simulink library "quatAttitudeController_lib"  (R2018b)
settings: Solver=VariableStepAuto  StartTime=0.0  StopTime=10.0  RelTol=1e-3
undefined symbols (not defined in the file or in its folder): quad
settings Model: Creator=fabian  LastModifiedBy=yannic

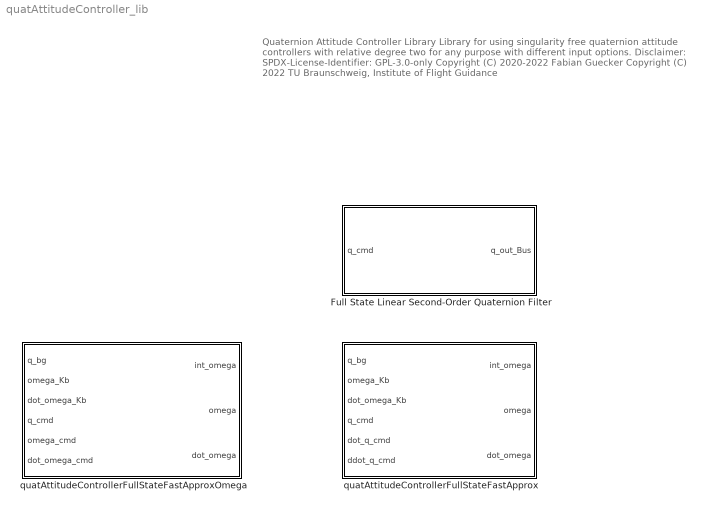
== system quatAttitudeController_lib ==
  note: Quaternion Attitude Controller Library
      |
      | Library for using singularity free quaternion attitude controllers with relative degree two
      | for any purpose with different input options.
      |
      | Disclaimer:
      | SPDX-License-Identifier: GPL-3.0-only
      |
      | Copyright (C) 2020-2022 Fabian Guecker
      | Copyright (C) 2022 TU Braunschweig, Institute of Flight Guidance
  Full State Linear Second-Order Quaternion Filter : Subsystem  mask{omega_0=200, D=1, q_0=[1; 0; 0; 0], omega_Kb_0=[0; 0; 0]}
      mask prompts: omega_0 "Natural frequency"; D "Damping factor"; q_0 "Inital quaternion"; omega_Kb_0 "Inital angular velocity"
  quatAttitudeControllerFullStateFastApprox : MATLAB Function  TreatAsAtomicUnit=on
  quatAttitudeControllerFullStateFastApproxOmega : MATLAB Function  TreatAsAtomicUnit=on

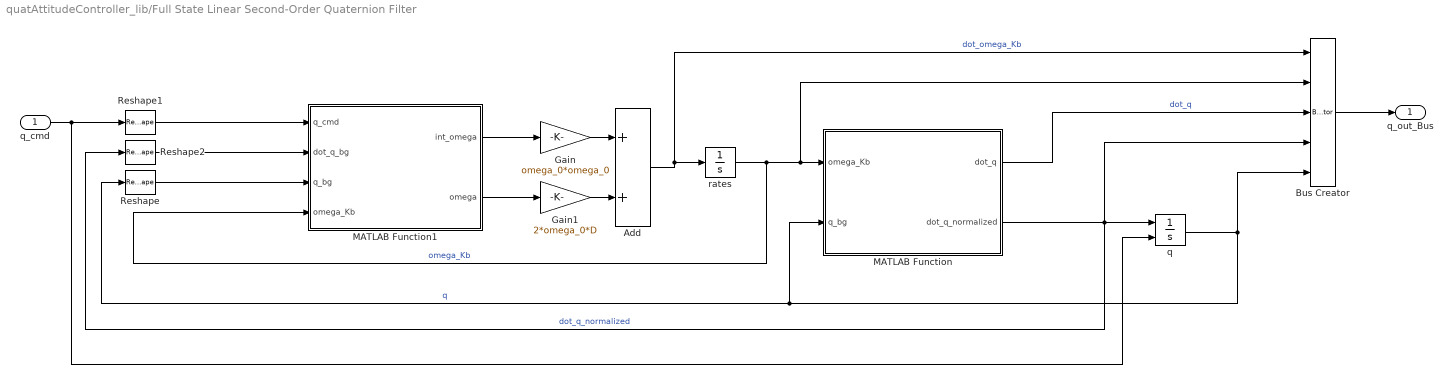
== system quatAttitudeController_lib/Full State Linear Second-Order Quaternion Filter ==
  q_cmd : Inport
  Add : Sum
  Bus Creator : BusCreator  Inputs=5
  Gain : Gain  Gain=omega_0*omega_0
  Gain1 : Gain  Gain=2*omega_0*D
  MATLAB Function : MATLAB Function  TreatAsAtomicUnit=on
  MATLAB Function1 : MATLAB Function  TreatAsAtomicUnit=on
  Reshape : Reshape  OutputDimensionality=Column vector (2-D)
  Reshape1 : Reshape  OutputDimensionality=Column vector (2-D)
  Reshape2 : Reshape  OutputDimensionality=Column vector (2-D)
  q : Integrator  InitialConditionSource=external  InitialCondition=q_0  UpperSaturationLimit=[inf;inf;-quad.z_s]  LowerSaturationLimit=[-inf;-inf;-inf]  ContinuousStateAttributes='quaternion'
  rates : Integrator  InitialCondition=omega_Kb_0  ContinuousStateAttributes='rates'
  q_out_Bus : Outport
  wires:
  Reshape/1 -> MATLAB Function1/3(q_bg)
  Reshape2/1 -> MATLAB Function1/2(dot_q_bg)
  Reshape1/1 -> MATLAB Function1/1(q_cmd)
  MATLAB Function1/2(omega) -> Gain1/1
  MATLAB Function1/1(int_omega) -> Gain/1
  q_cmd/1 -> Reshape1/1, q/2
  Gain/1 -> Add/1
  Gain1/1 -> Add/2
  rates/1 -> Bus Creator/2, MATLAB Function/1(omega_Kb), MATLAB Function1/4(omega_Kb)  "omega_Kb"
  q/1 -> Bus Creator/5, Reshape/1, MATLAB Function/2(q_bg)  "q"
  Add/1 -> rates/1, Bus Creator/1  "dot_omega_Kb"
  Bus Creator/1 -> q_out_Bus/1
  MATLAB Function/2(dot_q_normalized) -> Bus Creator/4, q/1, Reshape2/1  "dot_q_normalized"
  MATLAB Function/1(dot_q) -> Bus Creator/3  "dot_q"

== matlab function quatAttitudeController_lib/quatAttitudeControllerFullStateFastApproxOmega ==
  data: q_bg input; int_omega output; omega_Kb input; dot_omega_Kb input; q_cmd input; omega_cmd input; dot_omega_cmd input; omega output; dot_omega output
function [int_omega, omega, dot_omega] = fcn...
    (q_bg, omega_Kb, dot_omega_Kb, q_cmd, omega_cmd, dot_omega_cmd)

[int_omega, omega, dot_omega] = quatAttitudeControllerFullStateFastApproxOmega...
    (q_bg, omega_Kb, dot_omega_Kb, q_cmd, omega_cmd, dot_omega_cmd);

end

== matlab function quatAttitudeController_lib/quatAttitudeControllerFullStateFastApprox ==
  data: q_bg input; int_omega output; omega_Kb input; dot_omega_Kb input; q_cmd input; dot_q_cmd input; ddot_q_cmd input; omega output; dot_omega output
function [int_omega, omega, dot_omega] = fcn...
    (q_bg, omega_Kb, dot_omega_Kb, q_cmd, dot_q_cmd, ddot_q_cmd)

[int_omega, omega, dot_omega] = quatAttitudeControllerFullStateFastApprox...
    (q_bg, omega_Kb, dot_omega_Kb, q_cmd, dot_q_cmd, ddot_q_cmd);

end

== matlab function quatAttitudeController_lib/Full State Linear Second-Order Quaternion Filter/MATLAB Function ==
  data: omega_Kb input; dot_q output; q_bg input; dot_q_normalized output
function [dot_q, dot_q_normalized]   = ...
    rigidBodyKinematicsQuat( omega_Kb, q_bg )%#codegen

% compute the omega cross product matrix according to [1, page 8]
omega_cross_product = [ 0, omega_Kb(3), -omega_Kb(2); ...
                        -omega_Kb(3), 0, omega_Kb(1); ...
                        omega_Kb(2), -omega_Kb(1), 0 ];

% normalize quaternion
q_bg_norm = quatNormalize( q_bg );

% compute the time derivative of the quaternions vector according to
% [1, page 51]
dot_q = 0.5 * [ 0, -omega_Kb';...
                   omega_Kb, omega_cross_product ] ...
            * q_bg_norm;

% high gain quaternion normalization according to [2, page 3-60f]
k_quat = 1;
q_error = 1 - dot( q_bg, q_bg ); 
dot_q_normalized = dot_q + q_error * k_quat * q_bg_norm;


end

== matlab function quatAttitudeController_lib/Full State Linear Second-Order Quaternion Filter/MATLAB Function1 ==
  data: q_cmd input; dot_q_bg input; q_bg input; int_omega output; omega output; omega_Kb input
function [int_omega, omega] = quatAttitudeFilter...
    (q_cmd, dot_q_bg, q_bg, omega_Kb)

[int_omega, omega] = quatAttitudeFilter...
    (q_bg, dot_q_bg, q_cmd, omega_Kb);

end
